simulink model "motor_simulink"  (R2025b)
settings: Solver=FixedStepAuto  StartTime=0.0  StopTime=1  FixedStep=1e-4  RelTol=1e-3
undefined symbols (not defined in the file or in its folder): dspblkCoreblockFVToolHelper, gcbh
libraries: slpidlib x6, mcbplantlib x1, autolibpmsminterior x1
settings Model: Creator=wanghuixiang  LastModifiedBy=wanghuixiang

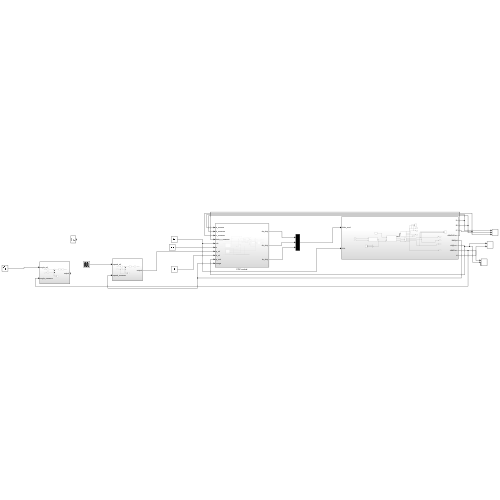
[thumbnail: Simulink's stored preview of the top-level diagram]
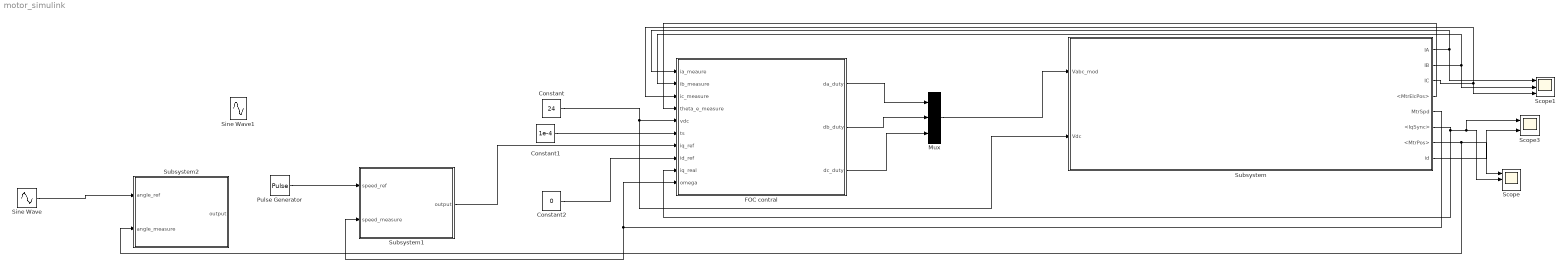
== system motor_simulink ==
  Constant : Constant  Value=24
  Constant1 : Constant  Value=1e-4
  Constant2 : Constant  Value=0
  FOC contral : Subsystem
  Mux : Mux  Inputs=3
  Pulse Generator : DiscretePulseGenerator  PulseType=Time based  Amplitude=30  Period=10  PulseWidth=5
  Scope : Scope  NumInputPorts=3
      settings: ActiveDisplayYMinimum=-4.2778704038949593  ActiveDisplayYMaximum=5.1731807364811857
  Scope1 : Scope  NumInputPorts=3
      settings: ActiveDisplayYMinimum=-271.31928354066577  ActiveDisplayYMaximum=293.76129527766454
  Scope3 : Scope  NumInputPorts=2
      settings: ActiveDisplayYMinimum=-0.10597587302872147  ActiveDisplayYMaximum=3.0541792317079626  DataLoggingVariableName=ScopeData9
  Sine Wave : Sin  Amplitude=0.5  Frequency=5  SampleTime=1e-4
  Sine Wave1 : Sin  Amplitude=50  Frequency=20  SampleTime=1e-4
  Subsystem : Subsystem
  Subsystem1 : Subsystem
  Subsystem2 : Subsystem
  wires:
  Constant/1 -> Subsystem/2(Vdc), FOC contral/5(vdc)
  Constant1/1 -> FOC contral/6(ts)
  FOC contral/1(da_duty) -> Mux/1
  FOC contral/2(db_duty) -> Mux/2
  FOC contral/3(dc_duty) -> Mux/3
  Subsystem/1(IA) -> Scope1/1, FOC contral/1(ia_meaure)
  Subsystem/3(IC) -> Scope1/3, FOC contral/3(ic_measure)
  Subsystem/2(IB) -> Scope1/2, FOC contral/2(ib_measure)
  Mux/1 -> Subsystem/1(Vabc_mod)
  Subsystem/6(<IqSync>) -> FOC contral/9(iq_real), Scope3/1, Scope/2
  Subsystem/7(<MtrPos>) -> Subsystem2/2(angle_measure), Scope/1
  Subsystem/8(id) -> Scope3/2
  Subsystem/4(<MtrElcPos>) -> FOC contral/4(theta_e_measure)
  Subsystem/5(MtrSpd) -> FOC contral/10(omega), Subsystem1/2(speed_measure)
  Sine Wave/1 -> Subsystem2/1(angle_ref)
  Constant2/1 -> FOC contral/8(id_ref)
  Subsystem1/1(output) -> FOC contral/7(iq_ref)
  Pulse Generator/1 -> Subsystem1/1(speed_ref)

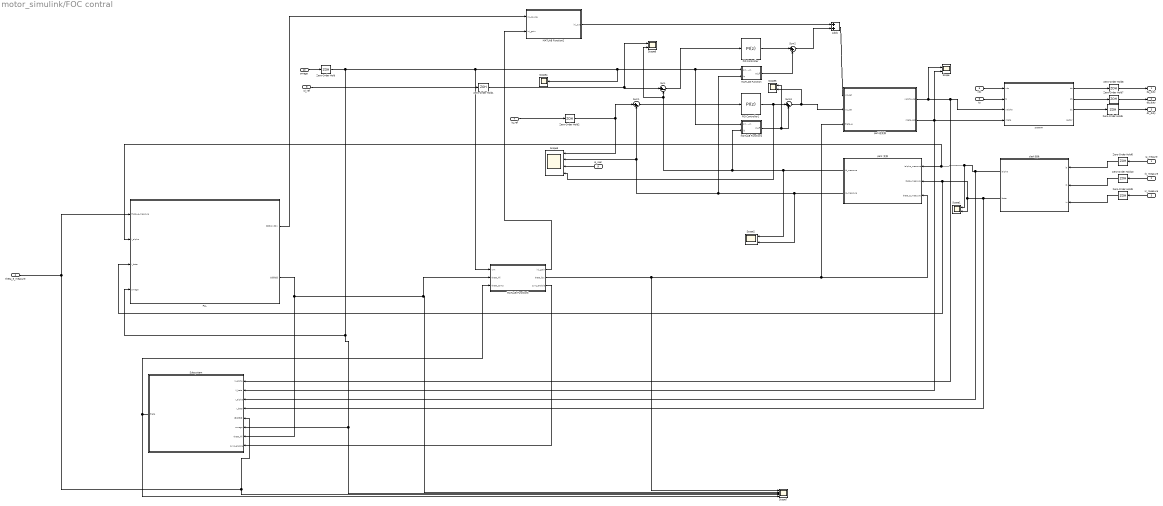
== system motor_simulink/FOC contral ==
  ia_meaure : Inport
  ib_measure : Inport  Port=2
  ic_measure : Inport  Port=3
  theta_e_measure : Inport  Port=4
  vdc : Inport  Port=5
  ts : Inport  Port=6
  iq_ref : Inport  Port=7
  id_ref : Inport  Port=8
  iq_real : Inport  Port=9
  omega : Inport  Port=10
  Add1 : Sum
  MATLAB Function : MATLAB Function  TreatAsAtomicUnit=on
  MATLAB Function1 : MATLAB Function  TreatAsAtomicUnit=on
  MATLAB Function2 : MATLAB Function  TreatAsAtomicUnit=on
  MATLAB Function3 : MATLAB Function  TreatAsAtomicUnit=on  SystemSampleTime=1e-4
  PID Controller : slpidlib/PID Controller  Controller=PI  Form=Parallel  TimeDomain=Discrete-time  UseExternalTs=off  SampleTime=1e-4  IntegratorMethod=Forward Euler  FilterMethod=Forward Euler  ControllerParametersSource=internal  P=0.2  I=0.0002  UseKiTs=on  D=0  UseExternalDerivativeSource=off  N=100  UseFilter=on  TunerSelectOption=Transfer Function Based (PID Tuner App)  InitialConditionSource=internal  InitialConditionForIntegrator=0  InitialConditionForFilter=0  DifferentiatorICPrevScaledInput=0  ExternalReset=none  TrackingMode=off  Kt=1  LimitOutput=on  SatLimitsSource=internal  UpperSaturationLimit=9.5  LowerSaturationLimit=-9.5  LinearizeAsGain=on  AntiWindupMode=none  Kb=1  LimitIntegrator=on  UpperIntegratorSaturationLimit=9.5  LowerIntegratorSaturationLimit=-9.5  POutMin=[]  POutMax=[]  IOutMin=[]  IOutMax=[]  DOutMin=[]  DOutMax=[]  NOutMin=[]  NOutMax=[]  SumOutMin=[]  SumOutMax=[]  SaturationOutMin=[]  SaturationOutMax=[]  PParamMin=[]  PParamMax=[]  IParamMin=[]  IParamMax=[]  DParamMin=[]  DParamMax=[]  NParamMin=[]  NParamMax=[]  KbParamMin=[]  KbParamMax=[]  KtParamMin=[]  KtParamMax=[]  KbOutMin=[]  KbOutMax=[]  KtOutMin=[]  KtOutMax=[]  IntegratorOutMin=[]  IntegratorOutMax=[]  FilterOutMin=[]  FilterOutMax=[]  SumI1OutMin=[]  SumI1OutMax=[]  SumI2OutMin=[]  SumI2OutMax=[]  SumI3OutMin=[]  SumI3OutMax=[]  SumI4OutMin=[]  SumI4OutMax=[]  SumDOutMin=[]  SumDOutMax=[]  DifferentiatorOutMin=[]  DifferentiatorOutMax=[]  FilterDiffOutCoefMin=[]  FilterDiffOutCoefMax=[]  ReciprocalOutMin=[]  ReciprocalOutMax=[]  SumDenOutMin=[]  SumDenOutMax=[]  SumNumOutMin=[]  SumNumOutMax=[]  DivideOutMin=[]  DivideOutMax=[]  UdiffTsProdOutMin=[]  UdiffTsProdOutMax=[]  NTsProdOutMin=[]  NTsProdOutMax=[]  UintegralTsProdOutMin=[]  UintegralTsProdOutMax=[]  UngainTsProdOutMin=[]  UngainTsProdOutMax=[]  ClampingZeroOutDataTypeStr=Inherit: Inherit via back propagation  ClampingZeroOutMin=[]  ClampingZeroOutMax=[]  FilterDenConstantOutDataTypeStr=Inherit: Inherit via back propagation  FilterDenConstantOutMin=[]  FilterDenConstantOutMax=[]  PCopyOutDataTypeStr=Inherit: Inherit via back propagation  PCopyOutMin=[]  PCopyOutMax=[]  NCopyOutDataTypeStr=Inherit: Inherit via back propagation  NCopyOutMin=[]  NCopyOutMax=[]  IntegratorContinuousStateAttributes=''  IntegratorStateMustResolveToSignalObject=off  IntegratorRTWStateStorageClass=Auto  FilterContinuousStateAttributes=''  FilterStateMustResolveToSignalObject=off  FilterRTWStateStorageClass=Auto  ParallelPVariant=InternalParameters  IdealPVariant=Disabled  IVariant=InternalParameters  DVariant=Disabled  IntegratorVariant=Discrete  SatVariant=Enabled  AWVariant=Passthrough  PCopyVariant=Disabled  TRVariant=Disabled  FdbkBlocksVariant=Forward  IdealPFdbkVariant=Disabled  SatFdbkVariant=Disabled  DerivativeFilterVariant=Disabled  NVariant=Disabled  NCopyVariant=Disabled_SignalSpec  FilterICVariant=Disabled  IntegratorICVariant=InternalICs  ExternalResetVariant=Disabled  TRSumVariant=Passthrough  SumFdbkVariant=Disabled  SumVariant=Sum_PI  TsampFilterVariant=InternalTs  TsampNgainVariant=Passthrough  TsampIntegralVariant=Disabled_SignalSpec  ExternalSaturationOutDataTypeStr=Inherit: Same as second input  DerivativeSourceVariant=Disabled  PreIntVariant=InternalPreInt
  PID Controller1 : slpidlib/PID Controller  Controller=PI  Form=Parallel  TimeDomain=Discrete-time  UseExternalTs=off  SampleTime=1e-4  IntegratorMethod=Forward Euler  FilterMethod=Forward Euler  ControllerParametersSource=internal  P=0.2  I=0.05  UseKiTs=on  D=0  UseExternalDerivativeSource=off  N=100  UseFilter=on  TunerSelectOption=Transfer Function Based (PID Tuner App)  InitialConditionSource=internal  InitialConditionForIntegrator=0  InitialConditionForFilter=0  DifferentiatorICPrevScaledInput=0  ExternalReset=none  TrackingMode=off  Kt=1  LimitOutput=on  SatLimitsSource=internal  UpperSaturationLimit=9.5  LowerSaturationLimit=-9.5  LinearizeAsGain=on  AntiWindupMode=none  Kb=1  LimitIntegrator=on  UpperIntegratorSaturationLimit=9.5  LowerIntegratorSaturationLimit=-9.5  POutMin=[]  POutMax=[]  IOutMin=[]  IOutMax=[]  DOutMin=[]  DOutMax=[]  NOutMin=[]  NOutMax=[]  SumOutMin=[]  SumOutMax=[]  SaturationOutMin=[]  SaturationOutMax=[]  PParamMin=[]  PParamMax=[]  IParamMin=[]  IParamMax=[]  DParamMin=[]  DParamMax=[]  NParamMin=[]  NParamMax=[]  KbParamMin=[]  KbParamMax=[]  KtParamMin=[]  KtParamMax=[]  KbOutMin=[]  KbOutMax=[]  KtOutMin=[]  KtOutMax=[]  IntegratorOutMin=[]  IntegratorOutMax=[]  FilterOutMin=[]  FilterOutMax=[]  SumI1OutMin=[]  SumI1OutMax=[]  SumI2OutMin=[]  SumI2OutMax=[]  SumI3OutMin=[]  SumI3OutMax=[]  SumI4OutMin=[]  SumI4OutMax=[]  SumDOutMin=[]  SumDOutMax=[]  DifferentiatorOutMin=[]  DifferentiatorOutMax=[]  FilterDiffOutCoefMin=[]  FilterDiffOutCoefMax=[]  ReciprocalOutMin=[]  ReciprocalOutMax=[]  SumDenOutMin=[]  SumDenOutMax=[]  SumNumOutMin=[]  SumNumOutMax=[]  DivideOutMin=[]  DivideOutMax=[]  UdiffTsProdOutMin=[]  UdiffTsProdOutMax=[]  NTsProdOutMin=[]  NTsProdOutMax=[]  UintegralTsProdOutMin=[]  UintegralTsProdOutMax=[]  UngainTsProdOutMin=[]  UngainTsProdOutMax=[]  ClampingZeroOutDataTypeStr=Inherit: Inherit via back propagation  ClampingZeroOutMin=[]  ClampingZeroOutMax=[]  FilterDenConstantOutDataTypeStr=Inherit: Inherit via back propagation  FilterDenConstantOutMin=[]  FilterDenConstantOutMax=[]  PCopyOutDataTypeStr=Inherit: Inherit via back propagation  PCopyOutMin=[]  PCopyOutMax=[]  NCopyOutDataTypeStr=Inherit: Inherit via back propagation  NCopyOutMin=[]  NCopyOutMax=[]  IntegratorContinuousStateAttributes=''  IntegratorStateMustResolveToSignalObject=off  IntegratorRTWStateStorageClass=Auto  FilterContinuousStateAttributes=''  FilterStateMustResolveToSignalObject=off  FilterRTWStateStorageClass=Auto  ParallelPVariant=InternalParameters  IdealPVariant=Disabled  IVariant=InternalParameters  DVariant=Disabled  IntegratorVariant=Discrete  SatVariant=Enabled  AWVariant=Passthrough  PCopyVariant=Disabled  TRVariant=Disabled  FdbkBlocksVariant=Forward  IdealPFdbkVariant=Disabled  SatFdbkVariant=Disabled  DerivativeFilterVariant=Disabled  NVariant=Disabled  NCopyVariant=Disabled_SignalSpec  FilterICVariant=Disabled  IntegratorICVariant=InternalICs  ExternalResetVariant=Disabled  TRSumVariant=Passthrough  SumFdbkVariant=Disabled  SumVariant=Sum_PI  TsampFilterVariant=InternalTs  TsampNgainVariant=Passthrough  TsampIntegralVariant=Disabled_SignalSpec  ExternalSaturationOutDataTypeStr=Inherit: Same as second input  DerivativeSourceVariant=Disabled  PreIntVariant=InternalPreInt
  PLL : Subsystem
  Scope{,1..2,5..6} (5 alike) : Scope  NumInputPorts=2
      Scope settings: ActiveDisplayYMinimum=-5.0548458842177206  ActiveDisplayYMaximum=5.2196458808879767  DataLoggingVariableName=ScopeData3
      Scope1 settings: ActiveDisplayYMinimum=-12.827305709885426  ActiveDisplayYMaximum=13.333371142328733  DataLoggingVariableName=ScopeData4
      Scope2 settings: ActiveDisplayYMinimum=-4.7470252065076783  ActiveDisplayYMaximum=4.9885520703342578  DataLoggingVariableName=ScopeData5
      Scope5 settings: ActiveDisplayYMinimum=-15.15417131801717  ActiveDisplayYMaximum=6.09591413502894  DataLoggingVariableName=ScopeData11
      Scope6 settings: ActiveDisplayYMinimum=-2.3979410109539563  ActiveDisplayYMaximum=4.879278024739981  DataLoggingVariableName=ScopeData13
  Scope3 : Scope  NumInputPorts=4
      settings: ActiveDisplayYMinimum=-4.5965064609442381  ActiveDisplayYMaximum=10.286487736088882  DataLoggingVariableName=ScopeData8
  Scope4 : Scope
      settings: ActiveDisplayYMinimum=-57.776270543491478  ActiveDisplayYMaximum=22.050412407087467  DataLoggingVariableName=ScopeData10
  Scope7 : Scope  NumInputPorts=5
      settings: ActiveDisplayYMinimum=-0.912671134531875  ActiveDisplayYMaximum=6.9599339439947947  DataLoggingVariableName=ScopeData15
  Subsystem : Subsystem
  Sum : Sum  Inputs=|+-
  Sum1 : Sum  Inputs=|+-
  Sum2 : Sum  Inputs=|++
  Sum3 : Sum  Inputs=|++
  Zero-Order Hold{,1..2,5..10} (9 alike) : ZeroOrderHold  SampleTime=1e-4
  clerk变换 : MATLAB Function  TreatAsAtomicUnit=on
  park 变换 : MATLAB Function  TreatAsAtomicUnit=on
  park逆变换 : MATLAB Function  TreatAsAtomicUnit=on
  svpwm : MATLAB Function  TreatAsAtomicUnit=on
  da_duty : Outport
  db_duty : Outport  Port=2
  dc_duty : Outport  Port=3
  wires:
  clerk变换/1(ialpha) -> Scope1/1, PLL/2(I_alpha), park 变换/1(ialpha_measure), Subsystem/3(I_alpha)
  clerk变换/2(ibeta) -> Subsystem/4(I_beta), Scope1/2, PLL/3(I_beta), park 变换/2(ibeta_measure)
  park逆变换/1(valpha_set) -> Subsystem/1(V_alpha), svpwm/3(valpha), Scope/1
  park逆变换/2(vbeta_set) -> Subsystem/2(V_beta), svpwm/4(vbeta), Scope/2
  svpwm/1(da) -> Zero-Order Hold8/1
  svpwm/2(db) -> Zero-Order Hold7/1
  svpwm/3(dc) -> Zero-Order Hold5/1
  vdc/1 -> svpwm/1(vdc)
  ts/1 -> svpwm/2(ts)
  park 变换/1(id_measure) -> Scope2/1, MATLAB Function1/2(id), Scope6/2, Sum/2
  id_ref/1 -> Zero-Order Hold1/1
  Sum/1 -> PID Controller/1
  Sum1/1 -> PID Controller1/1
  park 变换/2(iq_measure) -> Scope2/2, MATLAB Function/2(iq), Sum1/2, Scope3/2
  ia_meaure/1 -> Zero-Order Hold6/1
  ib_measure/1 -> Zero-Order Hold10/1
  ic_measure/1 -> Zero-Order Hold9/1
  iq_real/1 -> Scope3/3
  PID Controller/1 -> Sum2/1
  MATLAB Function/1(Vd_ff) -> Sum2/2
  PID Controller1/1 -> Scope3/4, Sum3/1
  MATLAB Function1/1(Vq_ff) -> Scope5/1, Sum3/2
  Sum3/1 -> Scope5/2, park逆变换/2(vq_set)
  omega/1 -> Zero-Order Hold/1
  Zero-Order Hold/1 -> PLL/4(omega), Scope7/3, Subsystem/6(omega), MATLAB Function3/1(wm), Scope4/1, MATLAB Function/1(omega_m), MATLAB Function1/1(omega_m)
  Zero-Order Hold2/1 -> Sum1/1, Scope3/1
  Zero-Order Hold6/1 -> clerk变换/1(ia)
  Zero-Order Hold10/1 -> clerk变换/2(ib)
  Zero-Order Hold9/1 -> clerk变换/3(ic)
  Zero-Order Hold8/1 -> da_duty/1
  Zero-Order Hold7/1 -> db_duty/1
  Zero-Order Hold5/1 -> dc_duty/1
  Sum2/1 -> Add1/2
  Add1/1 -> park逆变换/1(vd_set)
  theta_e_measure/1 -> Subsystem/5(真实角度), Scope7/4, PLL/1(theta_e_measure)
  iq_ref/1 -> Zero-Order Hold2/1
  Zero-Order Hold1/1 -> Sum/1, Scope6/1
  PLL/2(估算角度) -> Subsystem/7(theta_hfi), Scope7/2, MATLAB Function3/2(theta_hfi)
  Subsystem/1(theta) -> MATLAB Function3/3(theta_comp), Scope7/5
  MATLAB Function3/3(sync_enable) -> Subsystem/8(sync_enable)
  MATLAB Function3/1(inj_gain) -> MATLAB Function2/2(inj_gain)
  PLL/1(高频注入输入) -> MATLAB Function2/1(inj_source)
  MATLAB Function3/2(theta_foc) -> park逆变换/3(theta_e), park 变换/3(theta_e_measure), Scope7/1
  MATLAB Function2/1(inj_out) -> Add1/1

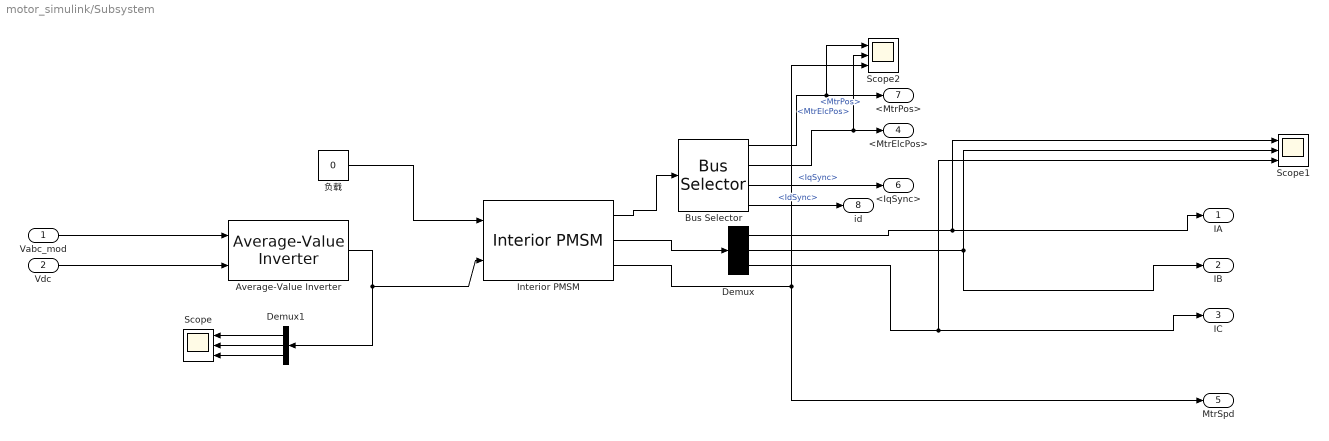
== system motor_simulink/Subsystem ==
  Vabc_mod : Inport
  Vdc : Inport  Port=2
  Average-Value Inverter : mcbplantlib/Average-Value Inverter
      settings: LibrarySourceBlock=mcblib/Electrical Systems/Inverters/Average-Value Inverter
  Bus Selector : BusSelector  OutputSignals=MtrPos,MtrElcPos,IqSync,IdSync
  Demux : Demux  Outputs=3
  Demux1 : Demux  Outputs=3
  Interior PMSM : autolibpmsminterior/Interior PMSM  port_config=Torque  sim_type=Discrete  Ts=1e-4  P=7  Rs=0.194  Ldq=[9.7e-5, 1.2e-4]  KConstText=Permanent flux linkage constant (lambda_pm):  lambda_pm=0.0016  Ke=159.9771  mechanical=[5e-5, 1e-4, 0]  idq0=[0 0]  theta_init=0  omega_init=0  KConst=0.2205  lambda_pm_calc=0.2205  Kt=0.07  RefBlkName='autolibpmsminterior/Interior PMSM'  aMode=5
      settings: LibrarySourceBlock=mcblib/Electrical Systems/Motors/Interior PMSM
  Scope : Scope  NumInputPorts=3
      settings: ActiveDisplayYMinimum=-22.197081060992033  ActiveDisplayYMaximum=25.053319218494003  DataLoggingVariableName=ScopeData6
  Scope1 : Scope  NumInputPorts=3
      settings: ActiveDisplayYMinimum=-132.21503565487177  ActiveDisplayYMaximum=147.93902485959063  DataLoggingVariableName=ScopeData7
  Scope2 : Scope  NumInputPorts=3
      settings: ActiveDisplayYMinimum=-44.268401921851606  ActiveDisplayYMaximum=132.86648709610233  DataLoggingVariableName=ScopeData19
  负载 : Constant  Value=0
  IA : Outport
  IB : Outport  Port=2
  IC : Outport  Port=3
  <MtrElcPos> : Outport  Port=4
  MtrSpd : Outport  Port=5
  <IqSync> : Outport  Port=6
  <MtrPos> : Outport  Port=7
  id : Outport  Port=8
  wires:
  负载/1 -> Interior PMSM/1
  Interior PMSM/2 -> Demux/1
  Average-Value Inverter/1 -> Demux1/1, Interior PMSM/2
  Interior PMSM/1 -> Bus Selector/1
  Interior PMSM/3 -> Scope2/3, MtrSpd/1
  Bus Selector/1 -> <MtrPos>/1, Scope2/1  "<MtrPos>"
  Bus Selector/2 -> Scope2/2, <MtrElcPos>/1  "<MtrElcPos>"
  Demux/1 -> IA/1, Scope1/1
  Demux/2 -> IB/1, Scope1/2
  Demux/3 -> IC/1, Scope1/3
  Demux1/1 -> Scope/1
  Demux1/2 -> Scope/2
  Demux1/3 -> Scope/3
  Vabc_mod/1 -> Average-Value Inverter/1
  Vdc/1 -> Average-Value Inverter/2
  Bus Selector/3 -> <IqSync>/1  "<IqSync>"
  Bus Selector/4 -> id/1  "<IdSync>"

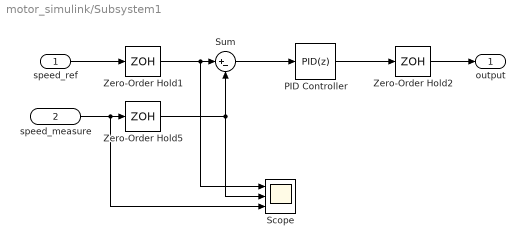
== system motor_simulink/Subsystem1 ==
  speed_ref : Inport
  speed_measure : Inport  Port=2
  PID Controller : slpidlib/PID Controller  Controller=PID  Form=Parallel  TimeDomain=Discrete-time  UseExternalTs=off  SampleTime=-1  IntegratorMethod=Forward Euler  FilterMethod=Forward Euler  ControllerParametersSource=internal  P=2  I=0  UseKiTs=on  D=0  UseExternalDerivativeSource=off  N=100  UseFilter=off  TunerSelectOption=Transfer Function Based (PID Tuner App)  InitialConditionSource=internal  InitialConditionForIntegrator=0  InitialConditionForFilter=0  DifferentiatorICPrevScaledInput=0  ExternalReset=none  TrackingMode=off  Kt=1  LimitOutput=on  SatLimitsSource=internal  UpperSaturationLimit=80  LowerSaturationLimit=-80  LinearizeAsGain=on  AntiWindupMode=none  Kb=1  LimitIntegrator=on  UpperIntegratorSaturationLimit=80  LowerIntegratorSaturationLimit=-80  POutMin=[]  POutMax=[]  IOutMin=[]  IOutMax=[]  DOutMin=[]  DOutMax=[]  NOutMin=[]  NOutMax=[]  SumOutMin=[]  SumOutMax=[]  SaturationOutMin=[]  SaturationOutMax=[]  PParamMin=[]  PParamMax=[]  IParamMin=[]  IParamMax=[]  DParamMin=[]  DParamMax=[]  NParamMin=[]  NParamMax=[]  KbParamMin=[]  KbParamMax=[]  KtParamMin=[]  KtParamMax=[]  KbOutMin=[]  KbOutMax=[]  KtOutMin=[]  KtOutMax=[]  IntegratorOutMin=[]  IntegratorOutMax=[]  FilterOutMin=[]  FilterOutMax=[]  SumI1OutMin=[]  SumI1OutMax=[]  SumI2OutMin=[]  SumI2OutMax=[]  SumI3OutMin=[]  SumI3OutMax=[]  SumI4OutMin=[]  SumI4OutMax=[]  SumDOutMin=[]  SumDOutMax=[]  DifferentiatorOutMin=[]  DifferentiatorOutMax=[]  FilterDiffOutCoefMin=[]  FilterDiffOutCoefMax=[]  ReciprocalOutMin=[]  ReciprocalOutMax=[]  SumDenOutMin=[]  SumDenOutMax=[]  SumNumOutMin=[]  SumNumOutMax=[]  DivideOutMin=[]  DivideOutMax=[]  UdiffTsProdOutMin=[]  UdiffTsProdOutMax=[]  NTsProdOutMin=[]  NTsProdOutMax=[]  UintegralTsProdOutMin=[]  UintegralTsProdOutMax=[]  UngainTsProdOutMin=[]  UngainTsProdOutMax=[]  ClampingZeroOutDataTypeStr=Inherit: Inherit via back propagation  ClampingZeroOutMin=[]  ClampingZeroOutMax=[]  FilterDenConstantOutDataTypeStr=Inherit: Inherit via back propagation  FilterDenConstantOutMin=[]  FilterDenConstantOutMax=[]  PCopyOutDataTypeStr=Inherit: Inherit via back propagation  PCopyOutMin=[]  PCopyOutMax=[]  NCopyOutDataTypeStr=Inherit: Inherit via back propagation  NCopyOutMin=[]  NCopyOutMax=[]  IntegratorContinuousStateAttributes=''  IntegratorStateMustResolveToSignalObject=off  IntegratorRTWStateStorageClass=Auto  FilterContinuousStateAttributes=''  FilterStateMustResolveToSignalObject=off  FilterRTWStateStorageClass=Auto  ParallelPVariant=InternalParameters  IdealPVariant=Disabled  IVariant=InternalParameters  DVariant=InternalParameters  IntegratorVariant=Discrete  SatVariant=Enabled  AWVariant=Passthrough  PCopyVariant=Disabled  TRVariant=Disabled  FdbkBlocksVariant=Forward  IdealPFdbkVariant=Disabled  SatFdbkVariant=Disabled  DerivativeFilterVariant=Differentiator  NVariant=Passthrough  NCopyVariant=Disabled_SignalSpec  FilterICVariant=InternalICsDifferentiator  IntegratorICVariant=InternalICs  ExternalResetVariant=Disabled  TRSumVariant=Passthrough  SumFdbkVariant=Disabled  SumVariant=Sum_PID  TsampFilterVariant=InternalTs  TsampNgainVariant=Passthrough  TsampIntegralVariant=Disabled_SignalSpec  ExternalSaturationOutDataTypeStr=Inherit: Same as second input  DerivativeSourceVariant=ErrorSignal  PreIntVariant=InternalPreInt
  Scope : Scope  NumInputPorts=3
      settings: ActiveDisplayYMinimum=-70.983114130808858  ActiveDisplayYMaximum=77.561026741553277  DataLoggingVariableName=ScopeData12
  Sum : Sum  Inputs=|+-
  Zero-Order Hold1 : ZeroOrderHold  SampleTime=1e-3
  Zero-Order Hold2 : ZeroOrderHold  SampleTime=1e-3
  Zero-Order Hold5 : ZeroOrderHold  SampleTime=1e-3
  output : Outport
  wires:
  speed_measure/1 -> Scope/3, Zero-Order Hold5/1
  speed_ref/1 -> Zero-Order Hold1/1
  Sum/1 -> PID Controller/1
  PID Controller/1 -> Zero-Order Hold2/1
  Zero-Order Hold2/1 -> output/1
  Zero-Order Hold1/1 -> Scope/1, Sum/1
  Zero-Order Hold5/1 -> Scope/2, Sum/2

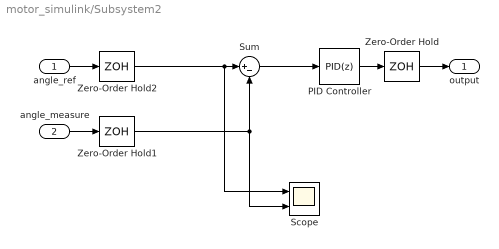
== system motor_simulink/Subsystem2 ==
  angle_ref : Inport
  angle_measure : Inport  Port=2
  PID Controller : slpidlib/PID Controller  Controller=PID  Form=Parallel  TimeDomain=Discrete-time  UseExternalTs=off  SampleTime=-1  IntegratorMethod=Forward Euler  FilterMethod=Forward Euler  ControllerParametersSource=internal  P=80  I=0  UseKiTs=on  D=0  UseExternalDerivativeSource=off  N=100  UseFilter=off  TunerSelectOption=Transfer Function Based (PID Tuner App)  InitialConditionSource=internal  InitialConditionForIntegrator=0  InitialConditionForFilter=0  DifferentiatorICPrevScaledInput=0  ExternalReset=none  TrackingMode=off  Kt=1  LimitOutput=on  SatLimitsSource=internal  UpperSaturationLimit=4000  LowerSaturationLimit=-4000  LinearizeAsGain=on  AntiWindupMode=none  Kb=1  LimitIntegrator=on  UpperIntegratorSaturationLimit=200  LowerIntegratorSaturationLimit=-200  POutMin=[]  POutMax=[]  IOutMin=[]  IOutMax=[]  DOutMin=[]  DOutMax=[]  NOutMin=[]  NOutMax=[]  SumOutMin=[]  SumOutMax=[]  SaturationOutMin=[]  SaturationOutMax=[]  PParamMin=[]  PParamMax=[]  IParamMin=[]  IParamMax=[]  DParamMin=[]  DParamMax=[]  NParamMin=[]  NParamMax=[]  KbParamMin=[]  KbParamMax=[]  KtParamMin=[]  KtParamMax=[]  KbOutMin=[]  KbOutMax=[]  KtOutMin=[]  KtOutMax=[]  IntegratorOutMin=[]  IntegratorOutMax=[]  FilterOutMin=[]  FilterOutMax=[]  SumI1OutMin=[]  SumI1OutMax=[]  SumI2OutMin=[]  SumI2OutMax=[]  SumI3OutMin=[]  SumI3OutMax=[]  SumI4OutMin=[]  SumI4OutMax=[]  SumDOutMin=[]  SumDOutMax=[]  DifferentiatorOutMin=[]  DifferentiatorOutMax=[]  FilterDiffOutCoefMin=[]  FilterDiffOutCoefMax=[]  ReciprocalOutMin=[]  ReciprocalOutMax=[]  SumDenOutMin=[]  SumDenOutMax=[]  SumNumOutMin=[]  SumNumOutMax=[]  DivideOutMin=[]  DivideOutMax=[]  UdiffTsProdOutMin=[]  UdiffTsProdOutMax=[]  NTsProdOutMin=[]  NTsProdOutMax=[]  UintegralTsProdOutMin=[]  UintegralTsProdOutMax=[]  UngainTsProdOutMin=[]  UngainTsProdOutMax=[]  ClampingZeroOutDataTypeStr=Inherit: Inherit via back propagation  ClampingZeroOutMin=[]  ClampingZeroOutMax=[]  FilterDenConstantOutDataTypeStr=Inherit: Inherit via back propagation  FilterDenConstantOutMin=[]  FilterDenConstantOutMax=[]  PCopyOutDataTypeStr=Inherit: Inherit via back propagation  PCopyOutMin=[]  PCopyOutMax=[]  NCopyOutDataTypeStr=Inherit: Inherit via back propagation  NCopyOutMin=[]  NCopyOutMax=[]  IntegratorContinuousStateAttributes=''  IntegratorStateMustResolveToSignalObject=off  IntegratorRTWStateStorageClass=Auto  FilterContinuousStateAttributes=''  FilterStateMustResolveToSignalObject=off  FilterRTWStateStorageClass=Auto  ParallelPVariant=InternalParameters  IdealPVariant=Disabled  IVariant=InternalParameters  DVariant=InternalParameters  IntegratorVariant=Discrete  SatVariant=Enabled  AWVariant=Passthrough  PCopyVariant=Disabled  TRVariant=Disabled  FdbkBlocksVariant=Forward  IdealPFdbkVariant=Disabled  SatFdbkVariant=Disabled  DerivativeFilterVariant=Differentiator  NVariant=Passthrough  NCopyVariant=Disabled_SignalSpec  FilterICVariant=InternalICsDifferentiator  IntegratorICVariant=InternalICs  ExternalResetVariant=Disabled  TRSumVariant=Passthrough  SumFdbkVariant=Disabled  SumVariant=Sum_PID  TsampFilterVariant=InternalTs  TsampNgainVariant=Passthrough  TsampIntegralVariant=Disabled_SignalSpec  ExternalSaturationOutDataTypeStr=Inherit: Same as second input  DerivativeSourceVariant=ErrorSignal  PreIntVariant=InternalPreInt
  Scope : Scope  NumInputPorts=2
      settings: ActiveDisplayYMinimum=-0.77126812647234222  ActiveDisplayYMaximum=1.1042710448596127  DataLoggingVariableName=ScopeData12
  Sum : Sum  Inputs=|+-
  Zero-Order Hold : ZeroOrderHold  SampleTime=0.01
  Zero-Order Hold1 : ZeroOrderHold  SampleTime=0.01
  Zero-Order Hold2 : ZeroOrderHold  SampleTime=0.01
  output : Outport
  wires:
  angle_measure/1 -> Zero-Order Hold1/1
  angle_ref/1 -> Zero-Order Hold2/1
  Sum/1 -> PID Controller/1
  PID Controller/1 -> Zero-Order Hold/1
  Zero-Order Hold2/1 -> Scope/1, Sum/1
  Zero-Order Hold1/1 -> Scope/2, Sum/2
  Zero-Order Hold/1 -> output/1

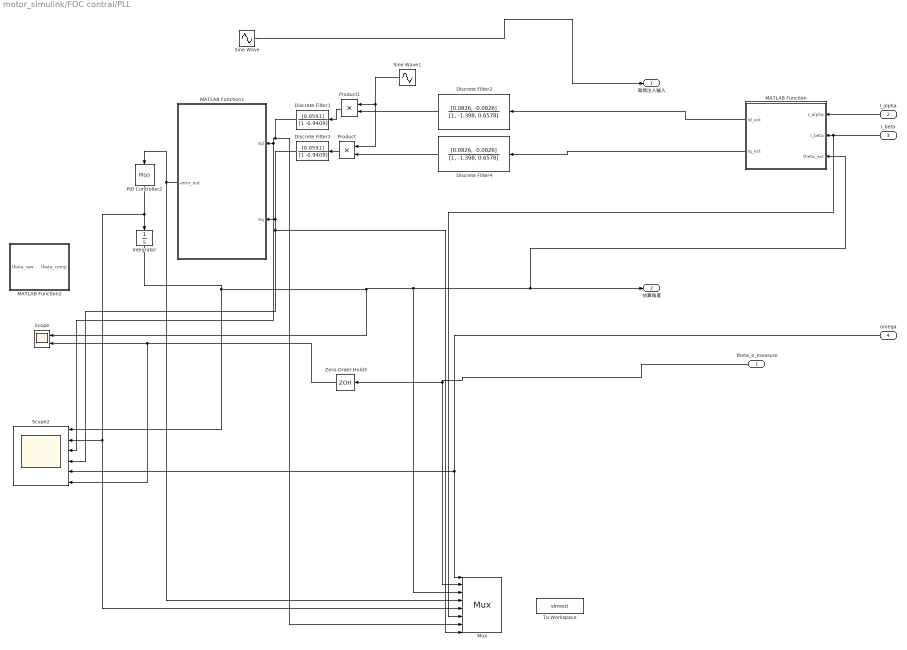
== system motor_simulink/FOC contral/PLL ==
  theta_e_measure : Inport
  I_alpha : Inport  Port=2
  I_beta : Inport  Port=3
  omega : Inport  Port=4
  Discrete Filter1 : DiscreteFilter  LoadFcn=dspblkCoreblockFVToolHelper(gcbh,'load');  Numerator=[0.0591]  Denominator=[1 -0.9409]
      settings: CopyFcn=dspblkCoreblockFVToolHelper(gcbh,'copy');  DeleteFcn=dspblkCoreblockFVToolHelper(gcbh,'close');  ModelCloseFcn=dspblkCoreblockFVToolHelper(gcbh,'close');  PreSaveFcn=dspblkCoreblockFVToolHelper(gcbh,'presave');  PostSaveFcn=dspblkCoreblockFVToolHelper(gcbh,'postsave');  CloseFcn=dspblkCoreblockFVToolHelper(gcbh,'close');
  Discrete Filter2 : DiscreteFilter  LoadFcn=dspblkCoreblockFVToolHelper(gcbh,'load');  Numerator=[0.0826, -0.0826]  Denominator=[1, -1.398, 0.6578]
      settings: CopyFcn=dspblkCoreblockFVToolHelper(gcbh,'copy');  DeleteFcn=dspblkCoreblockFVToolHelper(gcbh,'close');  ModelCloseFcn=dspblkCoreblockFVToolHelper(gcbh,'close');  PreSaveFcn=dspblkCoreblockFVToolHelper(gcbh,'presave');  PostSaveFcn=dspblkCoreblockFVToolHelper(gcbh,'postsave');  CloseFcn=dspblkCoreblockFVToolHelper(gcbh,'close');
  Discrete Filter3 : DiscreteFilter  LoadFcn=dspblkCoreblockFVToolHelper(gcbh,'load');  Numerator=[0.0591]  Denominator=[1 -0.9409]
      settings: CopyFcn=dspblkCoreblockFVToolHelper(gcbh,'copy');  DeleteFcn=dspblkCoreblockFVToolHelper(gcbh,'close');  ModelCloseFcn=dspblkCoreblockFVToolHelper(gcbh,'close');  PreSaveFcn=dspblkCoreblockFVToolHelper(gcbh,'presave');  PostSaveFcn=dspblkCoreblockFVToolHelper(gcbh,'postsave');  CloseFcn=dspblkCoreblockFVToolHelper(gcbh,'close');
  Discrete Filter4 : DiscreteFilter  LoadFcn=dspblkCoreblockFVToolHelper(gcbh,'load');  Numerator=[0.0826, -0.0826]  Denominator=[1, -1.398, 0.6578]
      settings: CopyFcn=dspblkCoreblockFVToolHelper(gcbh,'copy');  DeleteFcn=dspblkCoreblockFVToolHelper(gcbh,'close');  ModelCloseFcn=dspblkCoreblockFVToolHelper(gcbh,'close');  PreSaveFcn=dspblkCoreblockFVToolHelper(gcbh,'presave');  PostSaveFcn=dspblkCoreblockFVToolHelper(gcbh,'postsave');  CloseFcn=dspblkCoreblockFVToolHelper(gcbh,'close');
  Integrator : Integrator  WrapState=on  WrappedStateUpperValue=2*pi  WrappedStateLowerValue=0
  MATLAB Function : MATLAB Function  TreatAsAtomicUnit=on
  MATLAB Function1 : MATLAB Function  TreatAsAtomicUnit=on
  MATLAB Function2 : MATLAB Function  TreatAsAtomicUnit=on
  Mux : Mux  Inputs=8
  PID Controller2 : slpidlib/PID Controller  Controller=PI  Form=Parallel  TimeDomain=Discrete-time  UseExternalTs=off  SampleTime=1e-4  IntegratorMethod=Forward Euler  FilterMethod=Forward Euler  ControllerParametersSource=internal  P=1000  I=20  UseKiTs=on  D=0  UseExternalDerivativeSource=off  N=100  UseFilter=on  TunerSelectOption=Transfer Function Based (PID Tuner App)  InitialConditionSource=internal  InitialConditionForIntegrator=0  InitialConditionForFilter=0  DifferentiatorICPrevScaledInput=0  ExternalReset=none  TrackingMode=off  Kt=1  LimitOutput=off  SatLimitsSource=internal  UpperSaturationLimit=200  LowerSaturationLimit=-200  LinearizeAsGain=off  AntiWindupMode=none  Kb=1  LimitIntegrator=off  UpperIntegratorSaturationLimit=10  LowerIntegratorSaturationLimit=-10  POutMin=[]  POutMax=[]  IOutMin=[]  IOutMax=[]  DOutMin=[]  DOutMax=[]  NOutMin=[]  NOutMax=[]  SumOutMin=[]  SumOutMax=[]  SaturationOutMin=[]  SaturationOutMax=[]  PParamMin=[]  PParamMax=[]  IParamMin=[]  IParamMax=[]  DParamMin=[]  DParamMax=[]  NParamMin=[]  NParamMax=[]  KbParamMin=[]  KbParamMax=[]  KtParamMin=[]  KtParamMax=[]  KbOutMin=[]  KbOutMax=[]  KtOutMin=[]  KtOutMax=[]  IntegratorOutMin=[]  IntegratorOutMax=[]  FilterOutMin=[]  FilterOutMax=[]  SumI1OutMin=[]  SumI1OutMax=[]  SumI2OutMin=[]  SumI2OutMax=[]  SumI3OutMin=[]  SumI3OutMax=[]  SumI4OutMin=[]  SumI4OutMax=[]  SumDOutMin=[]  SumDOutMax=[]  DifferentiatorOutMin=[]  DifferentiatorOutMax=[]  FilterDiffOutCoefMin=[]  FilterDiffOutCoefMax=[]  ReciprocalOutMin=[]  ReciprocalOutMax=[]  SumDenOutMin=[]  SumDenOutMax=[]  SumNumOutMin=[]  SumNumOutMax=[]  DivideOutMin=[]  DivideOutMax=[]  UdiffTsProdOutMin=[]  UdiffTsProdOutMax=[]  NTsProdOutMin=[]  NTsProdOutMax=[]  UintegralTsProdOutMin=[]  UintegralTsProdOutMax=[]  UngainTsProdOutMin=[]  UngainTsProdOutMax=[]  ClampingZeroOutDataTypeStr=Inherit: Inherit via back propagation  ClampingZeroOutMin=[]  ClampingZeroOutMax=[]  FilterDenConstantOutDataTypeStr=Inherit: Inherit via back propagation  FilterDenConstantOutMin=[]  FilterDenConstantOutMax=[]  PCopyOutDataTypeStr=Inherit: Inherit via back propagation  PCopyOutMin=[]  PCopyOutMax=[]  NCopyOutDataTypeStr=Inherit: Inherit via back propagation  NCopyOutMin=[]  NCopyOutMax=[]  IntegratorContinuousStateAttributes=''  IntegratorStateMustResolveToSignalObject=off  IntegratorRTWStateStorageClass=Auto  FilterContinuousStateAttributes=''  FilterStateMustResolveToSignalObject=off  FilterRTWStateStorageClass=Auto  ParallelPVariant=InternalParameters  IdealPVariant=Disabled  IVariant=InternalParameters  DVariant=Disabled  IntegratorVariant=Discrete  SatVariant=Disabled  AWVariant=Passthrough  PCopyVariant=Disabled  TRVariant=Disabled  FdbkBlocksVariant=Forward  IdealPFdbkVariant=Disabled  SatFdbkVariant=Disabled  DerivativeFilterVariant=Disabled  NVariant=Disabled  NCopyVariant=Disabled_SignalSpec  FilterICVariant=Disabled  IntegratorICVariant=InternalICs  ExternalResetVariant=Disabled  TRSumVariant=Passthrough  SumFdbkVariant=Disabled  SumVariant=Sum_PI  TsampFilterVariant=InternalTs  TsampNgainVariant=Passthrough  TsampIntegralVariant=Disabled_SignalSpec  ExternalSaturationOutDataTypeStr=Inherit: Same as second input  DerivativeSourceVariant=Disabled  PreIntVariant=InternalPreInt
  Product : Product
  Product1 : Product
  Scope : Scope  NumInputPorts=2
      settings: ActiveDisplayYMinimum=-1.0258660467974963  ActiveDisplayYMaximum=7.3279003393936524  DataLoggingVariableName=ScopeData2
  Scope2 : Scope  NumInputPorts=6
      settings: ActiveDisplayYMinimum=-25.772472574684258  ActiveDisplayYMaximum=34.799963861540157  DataLoggingVariableName=ScopeData18
  Sine Wave : Sin  Amplitude=0.2  Frequency=6283  Phase=1.5708
  Sine Wave1 : Sin  Amplitude=0.2  Frequency=6283
  To Workspace : ToWorkspace  VariableName=simout  SaveFormat=Timeseries  SampleTime=1e-4
  Zero-Order Hold3 : ZeroOrderHold  SampleTime=1e-4
  高频注入输入 : Outport
  估算角度 : Outport  Port=2
  wires:
  theta_e_measure/1 -> Mux/2, Zero-Order Hold3/1
  Discrete Filter4/1 -> Product/2
  MATLAB Function1/1(error_out) -> Mux/4, PID Controller2/1
  Sine Wave/1 -> 高频注入输入/1
  PID Controller2/1 -> Mux/5, Scope2/2, Integrator/1
  Zero-Order Hold3/1 -> Scope2/6, Scope/2
  I_alpha/1 -> MATLAB Function/1(I_alpha)
  I_beta/1 -> Mux/6, MATLAB Function/2(I_beta)
  Sine Wave1/1 -> Product1/1, Product/1
  MATLAB Function/2(Iq_est) -> Discrete Filter4/1
  MATLAB Function/1(Id_est) -> Discrete Filter2/1
  Discrete Filter2/1 -> Product1/2
  Product1/1 -> Discrete Filter1/1
  Product/1 -> Discrete Filter3/1
  Discrete Filter1/1 -> Mux/7, Scope2/3, MATLAB Function1/1(Ed)
  Discrete Filter3/1 -> Scope2/4, Mux/8, MATLAB Function1/2(Eq)
  omega/1 -> Mux/1, Scope2/5
  Integrator/1 -> Scope2/1, Scope/1, MATLAB Function/3(theta_est), 估算角度/1, Mux/3

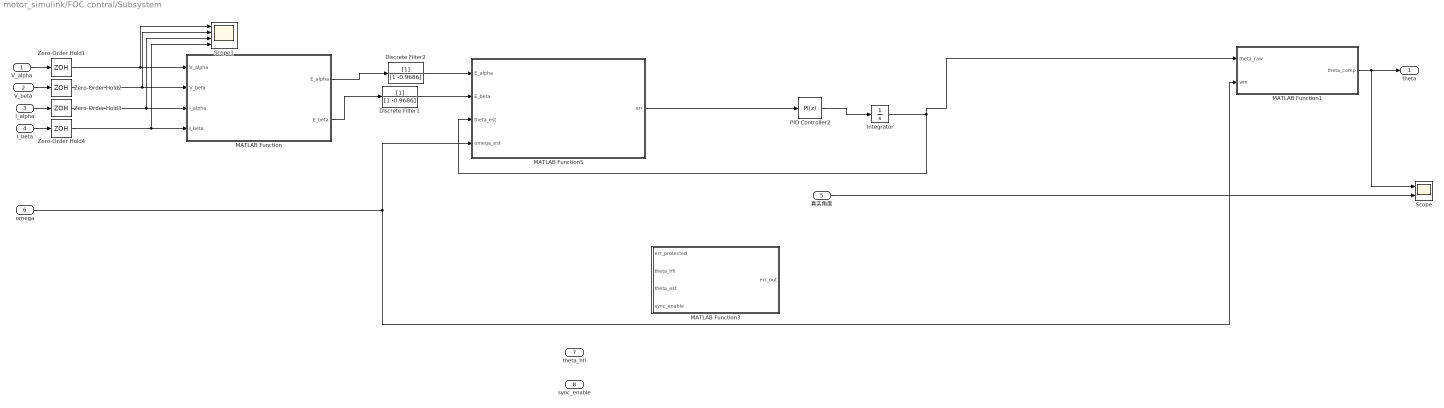
== system motor_simulink/FOC contral/Subsystem ==
  V_alpha : Inport
  V_beta : Inport  Port=2
  I_alpha : Inport  Port=3
  I_beta : Inport  Port=4
  真实角度 : Inport  Port=5
  omega : Inport  Port=6
  theta_hfi : Inport  Port=7
  sync_enable : Inport  Port=8
  Discrete Filter1 : DiscreteFilter  LoadFcn=dspblkCoreblockFVToolHelper(gcbh,'load');  Denominator=[1 -0.9686]
      settings: CopyFcn=dspblkCoreblockFVToolHelper(gcbh,'copy');  DeleteFcn=dspblkCoreblockFVToolHelper(gcbh,'close');  ModelCloseFcn=dspblkCoreblockFVToolHelper(gcbh,'close');  PreSaveFcn=dspblkCoreblockFVToolHelper(gcbh,'presave');  PostSaveFcn=dspblkCoreblockFVToolHelper(gcbh,'postsave');  CloseFcn=dspblkCoreblockFVToolHelper(gcbh,'close');
  Discrete Filter2 : DiscreteFilter  LoadFcn=dspblkCoreblockFVToolHelper(gcbh,'load');  Denominator=[1 -0.9686]
      settings: CopyFcn=dspblkCoreblockFVToolHelper(gcbh,'copy');  DeleteFcn=dspblkCoreblockFVToolHelper(gcbh,'close');  ModelCloseFcn=dspblkCoreblockFVToolHelper(gcbh,'close');  PreSaveFcn=dspblkCoreblockFVToolHelper(gcbh,'presave');  PostSaveFcn=dspblkCoreblockFVToolHelper(gcbh,'postsave');  CloseFcn=dspblkCoreblockFVToolHelper(gcbh,'close');
  Integrator : Integrator  WrapState=on  WrappedStateUpperValue=2*pi  WrappedStateLowerValue=0
  MATLAB Function : MATLAB Function  TreatAsAtomicUnit=on
  MATLAB Function1 : MATLAB Function  TreatAsAtomicUnit=on
  MATLAB Function3 : MATLAB Function  TreatAsAtomicUnit=on
  MATLAB Function5 : MATLAB Function  TreatAsAtomicUnit=on
  PID Controller2 : slpidlib/PID Controller  Controller=PI  Form=Parallel  TimeDomain=Discrete-time  UseExternalTs=off  SampleTime=1e-4  IntegratorMethod=Forward Euler  FilterMethod=Forward Euler  ControllerParametersSource=internal  P=15000  I=10  UseKiTs=on  D=0  UseExternalDerivativeSource=off  N=100  UseFilter=on  TunerSelectOption=Transfer Function Based (PID Tuner App)  InitialConditionSource=internal  InitialConditionForIntegrator=0  InitialConditionForFilter=0  DifferentiatorICPrevScaledInput=0  ExternalReset=none  TrackingMode=off  Kt=1  LimitOutput=off  SatLimitsSource=internal  UpperSaturationLimit=100  LowerSaturationLimit=-100  LinearizeAsGain=on  AntiWindupMode=none  Kb=1  LimitIntegrator=off  UpperIntegratorSaturationLimit=100  LowerIntegratorSaturationLimit=-100  POutMin=[]  POutMax=[]  IOutMin=[]  IOutMax=[]  DOutMin=[]  DOutMax=[]  NOutMin=[]  NOutMax=[]  SumOutMin=[]  SumOutMax=[]  SaturationOutMin=[]  SaturationOutMax=[]  PParamMin=[]  PParamMax=[]  IParamMin=[]  IParamMax=[]  DParamMin=[]  DParamMax=[]  NParamMin=[]  NParamMax=[]  KbParamMin=[]  KbParamMax=[]  KtParamMin=[]  KtParamMax=[]  KbOutMin=[]  KbOutMax=[]  KtOutMin=[]  KtOutMax=[]  IntegratorOutMin=[]  IntegratorOutMax=[]  FilterOutMin=[]  FilterOutMax=[]  SumI1OutMin=[]  SumI1OutMax=[]  SumI2OutMin=[]  SumI2OutMax=[]  SumI3OutMin=[]  SumI3OutMax=[]  SumI4OutMin=[]  SumI4OutMax=[]  SumDOutMin=[]  SumDOutMax=[]  DifferentiatorOutMin=[]  DifferentiatorOutMax=[]  FilterDiffOutCoefMin=[]  FilterDiffOutCoefMax=[]  ReciprocalOutMin=[]  ReciprocalOutMax=[]  SumDenOutMin=[]  SumDenOutMax=[]  SumNumOutMin=[]  SumNumOutMax=[]  DivideOutMin=[]  DivideOutMax=[]  UdiffTsProdOutMin=[]  UdiffTsProdOutMax=[]  NTsProdOutMin=[]  NTsProdOutMax=[]  UintegralTsProdOutMin=[]  UintegralTsProdOutMax=[]  UngainTsProdOutMin=[]  UngainTsProdOutMax=[]  ClampingZeroOutDataTypeStr=Inherit: Inherit via back propagation  ClampingZeroOutMin=[]  ClampingZeroOutMax=[]  FilterDenConstantOutDataTypeStr=Inherit: Inherit via back propagation  FilterDenConstantOutMin=[]  FilterDenConstantOutMax=[]  PCopyOutDataTypeStr=Inherit: Inherit via back propagation  PCopyOutMin=[]  PCopyOutMax=[]  NCopyOutDataTypeStr=Inherit: Inherit via back propagation  NCopyOutMin=[]  NCopyOutMax=[]  IntegratorContinuousStateAttributes=''  IntegratorStateMustResolveToSignalObject=off  IntegratorRTWStateStorageClass=Auto  FilterContinuousStateAttributes=''  FilterStateMustResolveToSignalObject=off  FilterRTWStateStorageClass=Auto  ParallelPVariant=InternalParameters  IdealPVariant=Disabled  IVariant=InternalParameters  DVariant=Disabled  IntegratorVariant=Discrete  SatVariant=Disabled  AWVariant=Passthrough  PCopyVariant=Disabled  TRVariant=Disabled  FdbkBlocksVariant=Forward  IdealPFdbkVariant=Disabled  SatFdbkVariant=Disabled  DerivativeFilterVariant=Disabled  NVariant=Disabled  NCopyVariant=Disabled_SignalSpec  FilterICVariant=Disabled  IntegratorICVariant=InternalICs  ExternalResetVariant=Disabled  TRSumVariant=Passthrough  SumFdbkVariant=Disabled  SumVariant=Sum_PI  TsampFilterVariant=InternalTs  TsampNgainVariant=Passthrough  TsampIntegralVariant=Disabled_SignalSpec  ExternalSaturationOutDataTypeStr=Inherit: Same as second input  DerivativeSourceVariant=Disabled  PreIntVariant=InternalPreInt
  Scope : Scope  NumInputPorts=2
      settings: ActiveDisplayYMinimum=-3.3948104569512179  ActiveDisplayYMaximum=12.186705937704335  DataLoggingVariableName=ScopeData14
  Scope1 : Scope  NumInputPorts=4
      settings: ActiveDisplayYMinimum=-7.72888363523471  ActiveDisplayYMaximum=8.4953267332173219  DataLoggingVariableName=ScopeData17
  Zero-Order Hold{1..4} (4 alike) : ZeroOrderHold  SampleTime=1e-4
  theta : Outport
  wires:
  I_alpha/1 -> Zero-Order Hold3/1
  V_beta/1 -> Zero-Order Hold2/1
  I_beta/1 -> Zero-Order Hold4/1
  V_alpha/1 -> Zero-Order Hold1/1
  Zero-Order Hold1/1 -> Scope1/1, MATLAB Function/1(V_alpha)
  Zero-Order Hold2/1 -> Scope1/2, MATLAB Function/2(V_beta)
  Zero-Order Hold3/1 -> Scope1/3, MATLAB Function/3(I_alpha)
  Zero-Order Hold4/1 -> Scope1/4, MATLAB Function/4(I_beta)
  PID Controller2/1 -> Integrator/1
  Integrator/1 -> MATLAB Function1/1(theta_raw), MATLAB Function5/3(theta_est)
  omega/1 -> MATLAB Function5/4(omega_est), MATLAB Function1/2(wm)
  MATLAB Function5/1(err) -> PID Controller2/1
  真实角度/1 -> Scope/2
  MATLAB Function/1(E_alpha) -> Discrete Filter2/1
  MATLAB Function/2(E_beta) -> Discrete Filter1/1
  Discrete Filter2/1 -> MATLAB Function5/1(E_alpha)
  Discrete Filter1/1 -> MATLAB Function5/2(E_beta)
  MATLAB Function1/1(theta_comp) -> Scope/1, theta/1

== matlab function motor_simulink/FOC contral/Subsystem/MATLAB Function3 ==
  data: err_protected input; err_out output; theta_hfi input; theta_est input; sync_enable input
function err_out = pre_sync_selector(err_protected, theta_hfi, theta_est, sync_enable)
    % 输入:
    %   err_protected: 磁观测原本算出的反电势误差
    %   theta_hfi:     高频注入输出的角度 (从图1引出)
    %   theta_est:     磁观测当前内部估计角度 (图2最下方积分器反馈回来的角度)
    %   sync_enable:   预同步使能信号 (来自顶层状态机)
    
    % 逻辑：如果 sync_enable > 0.5，强制跟随 HFI；否则正常使用反电势误差
    if sync_enable > 0.5
        % 计算强制跟随的误差
        err_out = sin(theta_hfi - theta_est);
    else
        % 正常情况
        err_out = err_protected;
    end
end

== matlab function motor_simulink/FOC contral/MATLAB Function2 ==
  data: inj_source input; inj_out output; inj_gain input
function inj_out = process_injection(inj_source, inj_gain)
    % 输入:
    %   inj_source: 原始的高频方波信号 (比如 ±Vh * sign(sin))
    %   inj_gain:   来自顶层状态机的注入增益 (正常为 1，关断为 0)
    % 输出:
    %   inj_out:    处理后的高频注入电压
    
    % 直接相乘：如果 inj_gain 为 0，则彻底切断注入
    inj_out = inj_source * inj_gain;
end

== matlab function motor_simulink/FOC contral/MATLAB Function3 ==
  data: inj_gain output; theta_foc output; wm input; theta_hfi input; theta_comp input; sync_enable output
function [inj_gain, theta_foc, sync_enable] = Supervisor_Final(wm, theta_hfi, theta_comp)
    abs_wm = abs(wm);
    
    % ==========================================
    % 1. 阈值设定 (机械速度 rad/s)
    % ==========================================
    W_inj_min  = 25; % 高于此值，维持微弱注入
    W_inj_max  = 15; % 低于此值，恢复满幅注入
    
    W_fuse_up  = 15; % 降速跌破此值，FOC 开始融合
    W_fuse_dn  = 8;  % 降速跌破此值，FOC 完全使用 HFI
    
    % ==========================================
    % 2. 注入幅值控制（保留微弱注入 -> 满幅预热）
    % ==========================================
    if abs_wm >= W_inj_min
        % 【高速区】：保留微弱注入，保证 HFI 的 PLL 一直有信号输入
        inj_gain = 0.3; 
        
    elseif abs_wm <= W_inj_max
        % 【低速区】：满幅注入，提供最高信噪比
        inj_gain = 1.0; 
        
    else
        % 【15 ~ 25 之间】：注入平滑从 0.3 渐变到 1.0
        % 这样不会因为突然增大幅值导致电流环突变
        ratio = (W_inj_min - abs_wm) / (W_inj_min - W_inj_max);
        inj_gain = 0.3 + ratio * 0.7;
    end
    
    % ==========================================
    % 3. 角度融合控制
    % ==========================================
    if abs_wm >= W_fuse_up
        % --- 高速及预热区（>15）：FOC 完全信任磁观测 ---
        % 此时 HFI 虽然活着，但因为在预热，角度可能还没完全收敛，坚决不用它！
        theta_foc = theta_comp;
        
    elseif abs_wm <= W_fuse_dn
        % --- 极低速区（<8）：FOC 完全信任 HFI ---
        theta_foc = theta_hfi;
        
    else
        % --- 融合区（8 ~ 15）：Sin/Cos 平滑加权 ---
        % alpha 从 0 (纯磁观测) 平滑过渡到 1 (纯 HFI)
        alpha = (W_fuse_up - abs_wm) / (W_fuse_up - W_fuse_dn);
        alpha = min(max(alpha, 0), 1); 
        
        s = alpha * sin(theta_hfi) + (1 - alpha) * sin(theta_comp);
        c = alpha * cos(theta_hfi) + (1 - alpha) * cos(theta_comp);
        theta_foc = atan2(s, c);
        theta_foc = mod(theta_foc, 2*pi);
    end
    
    % 不使用预同步
    sync_enable = 0; 
end

== matlab function motor_simulink/FOC contral/PLL/MATLAB Function ==
  data: I_alpha input; Id_est output; I_beta input; theta_est input; Iq_est output
function [Id_est, Iq_est] = HFI_Park(I_alpha, I_beta, theta_est)
    % 输入：I_alpha, I_beta (相电流)，theta_est (HFI内部估计角度)
    % 输出：用于解调的高频 d、q 轴电流
    
    % 标准双轴 Park 变换
    Id_est =  I_alpha * cos(theta_est) + I_beta * sin(theta_est);
    Iq_est = -I_alpha * sin(theta_est) + I_beta * cos(theta_est);
end

== matlab function motor_simulink/FOC contral/PLL/MATLAB Function1 ==
  data: Ed input; error_out output; Eq input
function error_out = HFI_Error_Calc(Ed, Eq)
    % 【核心修复】对输入信号进行硬限幅，削掉过零点的尖峰
    Ed_lim = max(min(Ed, 10), -10);
    Eq_lim = max(min(Eq, 10), -10);
    
    % 使用纯净的 atan2
    raw_error = atan2(Eq_lim, Ed_lim); 
    
    % 高频注入的 2 倍频特性
    error_out = raw_error / 2; 
end

== matlab function motor_simulink/FOC contral/Subsystem/MATLAB Function5 ==
  data: E_alpha input; err output; E_beta input; theta_est input; omega_est input
function err = calc_Angle_Error(E_alpha, E_beta, theta_est, omega_est)
    % 1. 计算反电动势幅值
    E_mag = sqrt(E_alpha^2 + E_beta^2);
    
    % 2. 低速死区保护 (防止静止或极低速时反电势过小导致误差乱跳)
    if E_mag < 0.05
        err = 0;
    else
        % 3. 计算原始误差 (反电势叉乘)
        err_raw = -E_alpha * cos(theta_est) - E_beta * sin(theta_est);
        
        % 4. 归一化 (把误差限制在 -1 到 1 之间，方便调 PI)
        err_norm = err_raw / E_mag; 
        
        % 5. 反转极性修正 (带死区)
        % 如果电机在正转，s=1；如果反转，s=-1；如果在零速附近，s=0
        if omega_est > 1.0
            s = 1;
        elseif omega_est < -1.0
            s = -1;
        else
            s = 0; 
        end
        
        err = err_norm * s;
    end
end

== matlab function motor_simulink/FOC contral/park逆变换 ==
  data: vd_set input; valpha_set output; vq_set input; theta_e input; vbeta_set output
function [valpha_set, vbeta_set] = inv_park_transform(vd_set, vq_set, theta_e)
    c = cos(theta_e);
    s = sin(theta_e);
    valpha_set = c*vd_set - s*vq_set;
    vbeta_set  = s*vd_set + c*vq_set;
end

== matlab function motor_simulink/FOC contral/park 变换 ==
  data: ialpha_measure input; id_measure output; ibeta_measure input; theta_e_measure input; iq_measure output
function [id_measure, iq_measure] = park_transform(ialpha_measure, ibeta_measure, theta_e_measure)
% Park 变换（等幅值）
% 输入：
%   ialpha, ibeta : α-β 轴电流
%   theta_e       : 电角度（rad）
% 输出：
%   id, iq        : d-q 轴电流
    c = cos(theta_e_measure);
    s = sin(theta_e_measure);
    id_measure =  c*ialpha_measure + s*ibeta_measure;
    iq_measure = -s*ialpha_measure + c*ibeta_measure;
end

== matlab function motor_simulink/FOC contral/clerk变换 ==
  data: ia input; ialpha output; ib input; ibeta output; ic input
function [ialpha, ibeta] = clarke_transform(ia, ib, ic)
% Clarke 正变换（等幅值）
% 输入：ia, ib, ic (三相电流)
% 输出：ialpha, ibeta
% 注意：默认 ia + ib + ic = 0
    
    ialpha = ia;
    ibeta = (1/sqrt(3)) * (ia + 2*ib); 
    % 或者写成：ibeta = (1/sqrt(3)) * (ib - ic);
    % 两者在 ia+ib+ic=0 时完全等价
end

== matlab function motor_simulink/FOC contral/svpwm ==
  data: vdc input; ts input; valpha input; da output; vbeta input; db output; dc output; sector output
function [da, db, dc, sector] = svpwm( vdc, ts,valpha, vbeta)
%#codegen
% SVPWM（七段式，中心对齐）
% 输入：valpha, vbeta —— 等幅值 Clarke 下的相电压给定
%       vdc           —— 母线电压
%       ts            —— PWM 周期
% 输出：da, db, dc    —— 三相占空比 [0,1]
%       sector        —— 当前扇区（调试用）

    if vdc < 1e-6
        vdc = 1e-6;
    end

    % ---------- 1. 扇区判断 ----------
    vref1 = vbeta;
    vref2 = 0.5*(sqrt(3)*valpha - vbeta);
    vref3 = 0.5*(-sqrt(3)*valpha - vbeta);

    A = vref1 > 0;
    B = vref2 > 0;
    C = vref3 > 0;
    N = A + 2*B + 4*C;

    switch N
        case 3, sector = 1;
        case 1, sector = 2;
        case 5, sector = 3;
        case 4, sector = 4;
        case 6, sector = 5;
        case 2, sector = 6;
        otherwise, sector = 1;   % N=0/7，零矢量附近，兜底
    end

    % ---------- 2. 中间变量 ----------
    X = sqrt(3)*ts*vbeta / vdc;
    Y = ts*(1.5*valpha + 0.5*sqrt(3)*vbeta) / vdc;
    Z = ts*(-1.5*valpha + 0.5*sqrt(3)*vbeta) / vdc;

    % ---------- 3. 作用时间 ----------
    switch sector
        case 1, T1 = -Z; T2 =  X;
        case 2, T1 =  Z; T2 =  Y;
        case 3, T1 =  X; T2 = -Y;
        case 4, T1 = -X; T2 =  Z;
        case 5, T1 = -Y; T2 = -Z;
        case 6, T1 =  Y; T2 = -X;
        otherwise, T1 = 0; T2 = 0;
    end

    % ---------- 4. 过调制限幅 ----------
    if (T1 + T2) > ts
        k  = ts / (T1 + T2);
        T1 = T1 * k;
        T2 = T2 * k;
    end
    if T1 < 0, T1 = 0; end
    if T2 < 0, T2 = 0; end

    % ---------- 5. 切换时间 ----------
    Ta = (ts - T1 - T2) / 4;
    Tb = Ta + T1/2;
    Tc = Tb + T2/2;

    switch sector
        case 1, Tcm1=Ta; Tcm2=Tb; Tcm3=Tc;
        case 2, Tcm1=Tb; Tcm2=Ta; Tcm3=Tc;
        case 3, Tcm1=Tc; Tcm2=Ta; Tcm3=Tb;
        case 4, Tcm1=Tc; Tcm2=Tb; Tcm3=Ta;
        case 5, Tcm1=Tb; Tcm2=Tc; Tcm3=Ta;
        case 6, Tcm1=Ta; Tcm2=Tc; Tcm3=Tb;
        otherwise, Tcm1=Ta; Tcm2=Tb; Tcm3=Tc;
    end

    % ---------- 6. 占空比计算 (已修正) ----------
    % 因为 Tcm 是低电平/零矢量的半周期时间，所以高电平占空比为 1 - 2 * (Tcm/ts)
    da = 1 - 2 * (Tcm1 / ts);
    db = 1 - 2 * (Tcm2 / ts);
    dc = 1 - 2 * (Tcm3 / ts);
end

== matlab function motor_simulink/FOC contral/MATLAB Function ==
  data: omega_m input; Vd_ff output; iq input
function Vd_ff = d_axis_ff(omega_m, iq)
    % --- 新电机参数 (与模型完全对齐) ---
    P = 7;              % 极对数
    Lq = 1.2e-4;        % q轴电感 (H) <- 【修正：原来是1.5e-5，改为与电机模型一致】
    
    % 计算电角速度
    omega_e = omega_m * P;
    
    % 理论交叉解耦前馈电压
    Vd_ff_raw = -omega_e * Lq * iq;
    
    % --- 防震荡平滑死区 ---
    weight = 1;
    % 输出平滑后的前馈电压
    Vd_ff = Vd_ff_raw * weight;
end

== matlab function motor_simulink/FOC contral/MATLAB Function1 ==
  data: omega_m input; Vq_ff output; id input
function Vq_ff = q_axis_ff(omega_m, id)
    % --- 新电机参数 (已同步修改) ---
    P = 7;              % 极对数
    Ld = 9.7e-5;        % d轴电感 (H) <- 【修正：原来是1e-5，改为与电机模型一致】
    flux = 0.0016;      % 永磁体磁链 (Wb) <- 【修正：原来是0.0036，改为0.0029】
    
    % 计算电角速度
    omega_e = omega_m * P;
    
    % 理论前馈电压 (反电动势项 + 交叉解耦项)
    % 公式：Vq_ff = ωe * ψf + ωe * Ld * id
    Vq_ff_raw = omega_e * flux + omega_e * Ld * id;
    
    % --- 防震荡平滑死区 ---
    % 注：这里 weight = 1 没有任何平滑作用，如果你不需要随转速平滑渐变，可以删掉这两行。
    weight = 1;
    
    % 输出平滑后的前馈电压
    Vq_ff = Vq_ff_raw * weight;
end

== matlab function motor_simulink/FOC contral/PLL/MATLAB Function2 ==
  data: theta_raw input; theta_comp output
function theta_comp = phase_compensation_hfi(theta_raw)
    Ts = 1e-4;
    a = 0.9686; % 你滤波器的极点
    Wh = 2 * pi * 1000; % 注入频率
    
    % 1. 计算固定相移角度 (这就是你说的限位频率的角度)
    lag_fixed = atan2(a * sin(Wh * Ts), 1 - a * cos(Wh * Ts));
    
    % 2. 因为你可能有多个滤波器 (BPF, LPF)，相移会叠加。
    % 假设你有两个这种滤波器，相移就是 2 * lag_fixed。
    % 根据你的实际波形，乘上一个校准系数（类似磁观测的 0.85）
    lag_final = lag_fixed * 1.0; 
    
    % 3. 直接补偿到角度上
    theta_comp = theta_raw + lag_final;
    theta_comp = mod(theta_comp, 2*pi);
end

== matlab function motor_simulink/FOC contral/Subsystem/MATLAB Function ==
  data: V_alpha input; E_alpha output; V_beta input; I_alpha input; I_beta input; E_beta output
function [E_alpha, E_beta] = calc_BEMF(V_alpha, V_beta, I_alpha, I_beta)
    % 电机参数直接写死
    Rs = 0.194; % 定子电阻 (Ohm)
    
    % 计算反电势原始值 (不含电感压降，因为中高速下感抗压降相对较小，且纯代数求导易受噪声干扰)
    E_alpha = V_alpha - Rs * I_alpha;
    E_beta  = V_beta  - Rs * I_beta;
end

== matlab function motor_simulink/FOC contral/Subsystem/MATLAB Function1 ==
  data: theta_raw input; wm input; theta_comp output
function theta_comp = phase_compensation_adaptive(theta_raw, wm)
    PolePairs = 7; 
    a = 0.9686; 
    Ts = 1e-4; % ！！！务必确认你的仿真步长！！！
    
    we = wm * PolePairs;
    abs_we = abs(we); 
    
    % 1. 理论滞后角
    lag_theory = atan2(a * sin(abs_we * Ts), 1 - a * cos(abs_we * Ts));
    lag_base = lag_theory * 0.85; % 基础校准
    
    % 2. 转速分段 (单位：电角速度 rad/s)
    we_start = 350; % 机械 50 rad/s
    we_mid = 560;   % 机械 80 rad/s
    we_end = 700;   % 机械 100 rad/s
    
    if abs_we <= we_start
        % 【中低速段】：50 rad/s 以下，全量补偿
        lag_final = lag_base; 
        
    elseif abs_we > we_start && abs_we <= we_mid
        % 【过渡段】：50 ~ 80 rad/s，从全量平滑降到 0.2
        lag_at_start = atan2(a * sin(we_start * Ts), 1 - a * cos(we_start * Ts)) * 0.85;
        ratio = (abs_we - we_start) / (we_mid - we_start);
        lag_final = lag_at_start - ratio * (lag_at_start - 0.2);
        
    elseif abs_we > we_mid && abs_we <= we_end
        % 【高速衰减段】：80 ~ 100 rad/s，从 0.2 平滑降到 0.1 (约5.7度)
        ratio = (abs_we - we_mid) / (we_end - we_mid);
        lag_final = 0.2 - ratio * 0.1; 
        
    else
        % 【极高速段】：> 100 rad/s，保留 0.1 的微弱补偿底线
        lag_final = 0.1; 
    end
    
    % 3. 赋予正负方向
    if we < 0
        lag_final = -lag_final; 
    end
    
    % 4. 应用补偿
    theta_comp = theta_raw + lag_final;
    theta_comp = mod(theta_comp, 2*pi);
end
